simulink model "mte484lab2parta"  (R2024a)
settings: Solver=VariableStepAuto  StartTime=0.0  StopTime=10.0  MaxStep=0.001  RelTol=1e-3
values from neighbouring files (symbols this model uses):
  A = 1.0    (= 1)    [mte484lab2asetup.m]
  Cden = [1 pc]    [mte484lab2asetup.m]
  Cnum = -k*[1 zc]    [mte484lab2asetup.m]
  freq = 0.5    [mte484lab2asetup.m]
  K1 = -1.883    [lab2a_data.mat]    (also in lab2b_data.mat; mte484lab2asetup.m)
  sat = 0.7    [mte484lab2asetup.m]
  tau = 0.0216    [lab2a_data.mat]    (also in lab2b_data.mat; mte484lab2asetup.m)
settings Model: Creator=christopherkoo  LastModifiedBy=christopherkoo

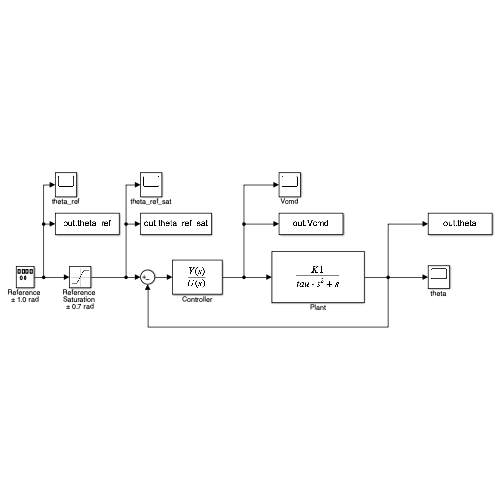
[thumbnail: Simulink's stored preview of the top-level diagram]
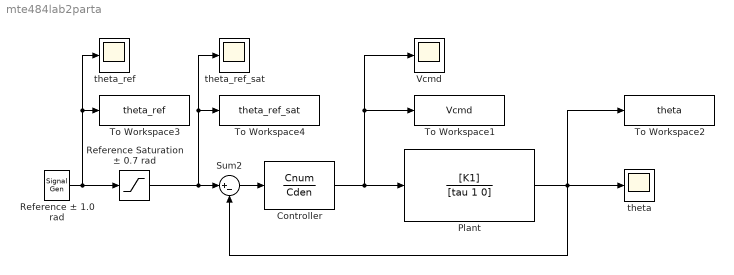
== system mte484lab2parta ==
  Controller : TransferFcn  Numerator=Cnum  Denominator=Cden
  Plant : TransferFcn  Numerator=[K1]  Denominator=[tau 1 0]
  Reference Saturation ± 0.7 rad : Saturate  UpperLimit=sat  LowerLimit=-sat
  Reference ± 1.0 rad : SignalGenerator  WaveForm=square  Amplitude=A  Frequency=freq
  Sum2 : Sum  Inputs=|+-
  To Workspace1 : ToWorkspace  VariableName=Vcmd  SaveFormat=Timeseries  SampleTime=-1
  To Workspace2 : ToWorkspace  VariableName=theta  SaveFormat=Timeseries  SampleTime=-1
  To Workspace3 : ToWorkspace  VariableName=theta_ref  SaveFormat=Timeseries  SampleTime=-1
  To Workspace4 : ToWorkspace  VariableName=theta_ref_sat  SaveFormat=Timeseries  SampleTime=-1
  Vcmd : Scope
  theta : Scope
  theta_ref : Scope
  theta_ref_sat : Scope
  wires:
  Controller/1 -> Plant/1, Vcmd/1, To Workspace1/1
  Plant/1 -> To Workspace2/1, theta/1, Sum2/2
  Sum2/1 -> Controller/1
  Reference Saturation ± 0.7 rad/1 -> theta_ref_sat/1, To Workspace4/1, Sum2/1
  Reference ± 1.0 rad/1 -> Reference Saturation ± 0.7 rad/1, theta_ref/1, To Workspace3/1
